simulink model "printable_simulation"  (R2024b)
settings: Solver=ode1be  StartTime=0.0  StopTime=10  FixedStep=0.001  RelTol=1e-3
model workspace (MAT data in the model file):
  AMP = 1
  FREQ = 1
  i_abc = 1
undefined symbols (not defined in the file or in its folder): Drive_wheel, Driveshaft, eff_shaft, f_OVD, i, J_S21, Jr2, K, M_curve_1, M_curve_2, M_total, mi_c, mi_s, Mode, N_clutch, n_curve_1, n_curve_2, n_max_1, n_max_2, n_surfaces, Pl, r_eq_clutch, r_geom, Shaft, sigma0, sigma1, sigma2, Spurs_Inertia, Stage1, Stage2, Stage3, vs, wheel_width
libraries: simulink x12, slpidlib x1
(part 2 of 3)

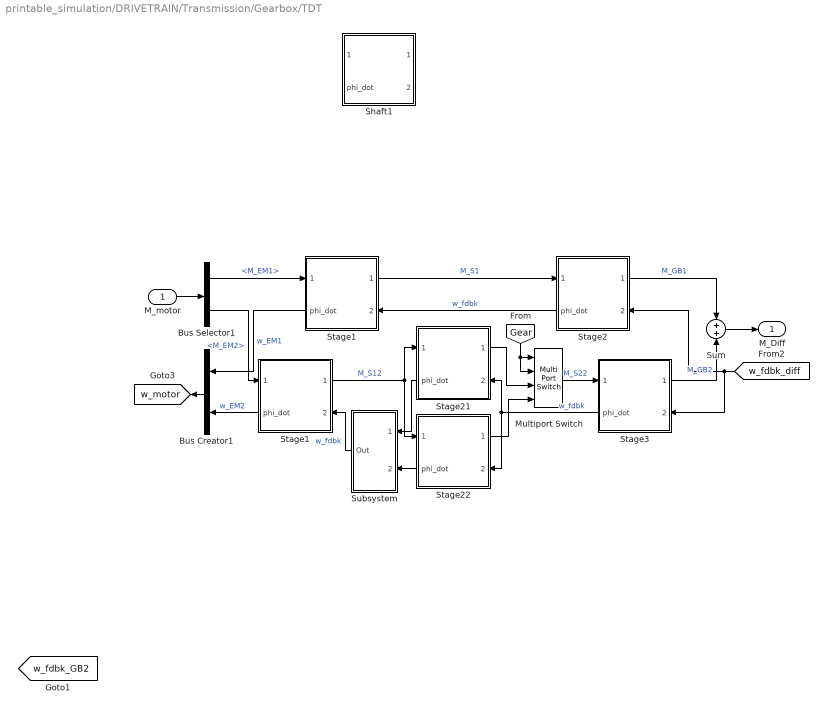
== system printable_simulation/DRIVETRAIN/Transmission/Gearbox/TDT ==
  M_motor : Inport
  Bus Creator1 : BusCreator  Inputs=2
  Bus Selector1 : BusSelector  OutputSignals=M_EM1,M_EM2
  Multiport Switch : MultiPortSwitch  DataPortOrder=Zero-based contiguous  zeroidx=on  SaturateOnIntegerOverflow=off  InputSameDT=off
  Shaft1 : Subsystem  mask{J=Shaft.J}
      mask prompts: J "Inertia_kgm^2"
      settings: PortSchema="{\"entries\":[{\"content\":{\"sides\":[{\"content\":{\"connectorIds\":[\"In1\",\"Out2\"]},\"type\":\"ConnectorPlacement.EquallySpacedRectSide\",\"uuid\":\"898fedf9-82f7-4bc2-bf05-880de36b191d\"},{\"content\":{\"connectorIds\":[\"Out1\",\"In2\"],\"side\":\"RIGHT\"},\"type\":\"ConnectorPlacement.EquallySpacedRectSide\",\"uuid\":\"50317b6c-245f-4bd1-a8cd-7a774957ae86\"},{\"content\":{\"side\":\"TOP\"},\"type\":\"ConnectorPlacement.EquallySpacedRectSide\",\"uuid\":\"ff1de2a1-7305-40d8-9e1f-fd0fa1e7d830\"}]},\"type\":\"ConnectorPlacement.EquallySpacedConnector\",\"uuid\":\"6ce82d73-f3da-4f59-9039-464a6ef3e9c5\"}],\"packageUris\":[\"http://schema.mathworks.com/mf0/Connector/R2020b\"],\"version\":\"1.0\"}"
  Stage1 : Subsystem  mask{i=Stage2.i1, J1=Stage2.Spur11.J, J2=Stage2.Spur12.J}
      mask prompts: i "Ratio"; J1 "Input_Gear_Inertia"; J2 "Output_Gear_Inertia"
      settings: PortSchema="{\"entries\":[{\"content\":{\"sides\":[{\"content\":{\"connectorIds\":[\"In1\",\"Out2\"]},\"type\":\"ConnectorPlacement.EquallySpacedRectSide\",\"uuid\":\"898fedf9-82f7-4bc2-bf05-880de36b191d\"},{\"content\":{\"connectorIds\":[\"Out1\",\"In2\"],\"side\":\"RIGHT\"},\"type\":\"ConnectorPlacement.EquallySpacedRectSide\",\"uuid\":\"50317b6c-245f-4bd1-a8cd-7a774957ae86\"},{\"content\":{\"side\":\"TOP\"},\"type\":\"ConnectorPlacement.EquallySpacedRectSide\",\"uuid\":\"ff1de2a1-7305-40d8-9e1f-fd0fa1e7d830\"}]},\"type\":\"ConnectorPlacement.EquallySpacedConnector\",\"uuid\":\"6ce82d73-f3da-4f59-9039-464a6ef3e9c5\"}],\"packageUris\":[\"http://schema.mathworks.com/mf0/Connector/R2020b\"],\"version\":\"1.0\"}"
      mask Display: image("images/spur_reduction.jpg");
  "Stage1 " : Subsystem  mask{i=Stage2.i1, J1=Stage2.Spur11.J, J2=Stage2.Spur12.J}
      mask prompts: i "Ratio"; J1 "Input_Gear_Inertia"; J2 "Output_Gear_Inertia"
      settings: PortSchema="{\"entries\":[{\"content\":{\"sides\":[{\"content\":{\"connectorIds\":[\"In1\",\"Out2\"]},\"type\":\"ConnectorPlacement.EquallySpacedRectSide\",\"uuid\":\"898fedf9-82f7-4bc2-bf05-880de36b191d\"},{\"content\":{\"connectorIds\":[\"Out1\",\"In2\"],\"side\":\"RIGHT\"},\"type\":\"ConnectorPlacement.EquallySpacedRectSide\",\"uuid\":\"50317b6c-245f-4bd1-a8cd-7a774957ae86\"},{\"content\":{\"side\":\"TOP\"},\"type\":\"ConnectorPlacement.EquallySpacedRectSide\",\"uuid\":\"ff1de2a1-7305-40d8-9e1f-fd0fa1e7d830\"}]},\"type\":\"ConnectorPlacement.EquallySpacedConnector\",\"uuid\":\"6ce82d73-f3da-4f59-9039-464a6ef3e9c5\"}],\"packageUris\":[\"http://schema.mathworks.com/mf0/Connector/R2020b\"],\"version\":\"1.0\"}"
      mask Display: image("images/spur_reduction.jpg");
  Stage2 : Subsystem  mask{i=Stage2.i1, J1=Stage2.Spur11.J, J2=Stage2.Spur12.J}
      mask prompts: i "Ratio"; J1 "Input_Gear_Inertia"; J2 "Output_Gear_Inertia"
      settings: PortSchema="{\"entries\":[{\"content\":{\"sides\":[{\"content\":{\"connectorIds\":[\"In1\",\"Out2\"]},\"type\":\"ConnectorPlacement.EquallySpacedRectSide\",\"uuid\":\"898fedf9-82f7-4bc2-bf05-880de36b191d\"},{\"content\":{\"connectorIds\":[\"Out1\",\"In2\"],\"side\":\"RIGHT\"},\"type\":\"ConnectorPlacement.EquallySpacedRectSide\",\"uuid\":\"50317b6c-245f-4bd1-a8cd-7a774957ae86\"},{\"content\":{\"side\":\"TOP\"},\"type\":\"ConnectorPlacement.EquallySpacedRectSide\",\"uuid\":\"ff1de2a1-7305-40d8-9e1f-fd0fa1e7d830\"}]},\"type\":\"ConnectorPlacement.EquallySpacedConnector\",\"uuid\":\"6ce82d73-f3da-4f59-9039-464a6ef3e9c5\"}],\"packageUris\":[\"http://schema.mathworks.com/mf0/Connector/R2020b\"],\"version\":\"1.0\"}"
      mask Display: image("images/spur_reduction.jpg");
  Stage21 : Subsystem  mask{i=Stage2.i1, J1=Stage2.Spur11.J, J2=Stage2.Spur12.J}
      mask prompts: i "Ratio"; J1 "Input_Gear_Inertia"; J2 "Output_Gear_Inertia"
      settings: PortSchema="{\"entries\":[{\"content\":{\"sides\":[{\"content\":{\"connectorIds\":[\"In1\",\"Out2\"]},\"type\":\"ConnectorPlacement.EquallySpacedRectSide\",\"uuid\":\"898fedf9-82f7-4bc2-bf05-880de36b191d\"},{\"content\":{\"connectorIds\":[\"Out1\",\"In2\"],\"side\":\"RIGHT\"},\"type\":\"ConnectorPlacement.EquallySpacedRectSide\",\"uuid\":\"50317b6c-245f-4bd1-a8cd-7a774957ae86\"},{\"content\":{\"side\":\"TOP\"},\"type\":\"ConnectorPlacement.EquallySpacedRectSide\",\"uuid\":\"ff1de2a1-7305-40d8-9e1f-fd0fa1e7d830\"}]},\"type\":\"ConnectorPlacement.EquallySpacedConnector\",\"uuid\":\"6ce82d73-f3da-4f59-9039-464a6ef3e9c5\"}],\"packageUris\":[\"http://schema.mathworks.com/mf0/Connector/R2020b\"],\"version\":\"1.0\"}"
      mask Display: image("images/spur_reduction.jpg");
  Stage22 : Subsystem  mask{i=Stage2.i1, J1=Stage2.Spur11.J, J2=Stage2.Spur12.J}
      mask prompts: i "Ratio"; J1 "Input_Gear_Inertia"; J2 "Output_Gear_Inertia"
      settings: PortSchema="{\"entries\":[{\"content\":{\"sides\":[{\"content\":{\"connectorIds\":[\"In1\",\"Out2\"]},\"type\":\"ConnectorPlacement.EquallySpacedRectSide\",\"uuid\":\"898fedf9-82f7-4bc2-bf05-880de36b191d\"},{\"content\":{\"connectorIds\":[\"Out1\",\"In2\"],\"side\":\"RIGHT\"},\"type\":\"ConnectorPlacement.EquallySpacedRectSide\",\"uuid\":\"50317b6c-245f-4bd1-a8cd-7a774957ae86\"},{\"content\":{\"side\":\"TOP\"},\"type\":\"ConnectorPlacement.EquallySpacedRectSide\",\"uuid\":\"ff1de2a1-7305-40d8-9e1f-fd0fa1e7d830\"}]},\"type\":\"ConnectorPlacement.EquallySpacedConnector\",\"uuid\":\"6ce82d73-f3da-4f59-9039-464a6ef3e9c5\"}],\"packageUris\":[\"http://schema.mathworks.com/mf0/Connector/R2020b\"],\"version\":\"1.0\"}"
      mask Display: image("images/spur_reduction.jpg");
  Stage3 : Subsystem  mask{i=Stage2.i1, J1=Stage2.Spur11.J, J2=Stage2.Spur12.J}
      mask prompts: i "Ratio"; J1 "Input_Gear_Inertia"; J2 "Output_Gear_Inertia"
      settings: PortSchema="{\"entries\":[{\"content\":{\"sides\":[{\"content\":{\"connectorIds\":[\"In1\",\"Out2\"]},\"type\":\"ConnectorPlacement.EquallySpacedRectSide\",\"uuid\":\"898fedf9-82f7-4bc2-bf05-880de36b191d\"},{\"content\":{\"connectorIds\":[\"Out1\",\"In2\"],\"side\":\"RIGHT\"},\"type\":\"ConnectorPlacement.EquallySpacedRectSide\",\"uuid\":\"50317b6c-245f-4bd1-a8cd-7a774957ae86\"},{\"content\":{\"side\":\"TOP\"},\"type\":\"ConnectorPlacement.EquallySpacedRectSide\",\"uuid\":\"ff1de2a1-7305-40d8-9e1f-fd0fa1e7d830\"}]},\"type\":\"ConnectorPlacement.EquallySpacedConnector\",\"uuid\":\"6ce82d73-f3da-4f59-9039-464a6ef3e9c5\"}],\"packageUris\":[\"http://schema.mathworks.com/mf0/Connector/R2020b\"],\"version\":\"1.0\"}"
      mask Display: image("images/spur_reduction.jpg");
  Subsystem : Subsystem
      settings: PortSchema="{\"entries\":[{\"content\":{\"sides\":[{\"content\":{\"connectorIds\":[\"Out1\"]},\"type\":\"ConnectorPlacement.EquallySpacedRectSide\",\"uuid\":\"fb6fb521-24b4-42a9-962b-0690c95a6555\"},{\"content\":{\"connectorIds\":[\"In1\",\"In2\"],\"side\":\"RIGHT\"},\"type\":\"ConnectorPlacement.EquallySpacedRectSide\",\"uuid\":\"05ff3728-9142-4ede-8c02-c3816594f1d6\"},{\"content\":{\"side\":\"TOP\"},\"type\":\"ConnectorPlacement.EquallySpacedRectSide\",\"uuid\":\"6bf5bb06-bb76-41b4-800b-6d1bd3df4c7c\"}]},\"type\":\"ConnectorPlacement.EquallySpacedConnector\",\"uuid\":\"4f0648fe-100b-4dfa-b2f8-0696c3f6a986\"}],\"packageUris\":[\"http://schema.mathworks.com/mf0/Connector/R2020b\"],\"version\":\"1.0\"}"
      mask Display: image("images/switch.png");
  Sum : Sum  Inputs=+|+
  M_Diff : Outport
  tag scope: w_fdbk_GB2=global, w_motor=global
  wires:
  "Stage1 "/1(Torque_out) -> Stage21/1(Torque_in), Stage22/1(Torque_in)  "M_S12"
  M_motor/1 -> Bus Selector1/1
  Stage3/1(Torque_out) -> Sum/2  "M_GB2"
  Bus Selector1/1 -> Stage1/1(Torque_in)  "<M_EM1>"
  Stage2/1(Torque_out) -> Sum/1  "M_GB1"
  Stage1/2(phi_dot) -> Bus Creator1/1  "w_EM1"
  Bus Selector1/2 -> "Stage1 "/1(Torque_in)  "<M_EM2>"
  Sum/1 -> M_Diff/1
  Stage1/1(Torque_out) -> Stage2/1(Torque_in)  "M_S1"
  Stage3/2(phi_dot) -> Stage22/2(Speed_fdbk), Stage21/2(Speed_fdbk)  "w_fdbk"
  Multiport Switch/1 -> Stage3/1(Torque_in)  "M_S22"
  Stage22/2(phi_dot) -> Subsystem/2(Spur22)
  [w_fdbk_diff] -> Stage2/2(Speed_fdbk), Stage3/2(Speed_fdbk)
  Stage22/1(Torque_out) -> Multiport Switch/4
  [Gear] -> Multiport Switch/1, Multiport Switch/2
  Stage21/2(phi_dot) -> Subsystem/1(Spur 21)
  "Stage1 "/2(phi_dot) -> Bus Creator1/2  "w_EM2"
  Bus Creator1/1 -> [w_motor]
  Stage21/1(Torque_out) -> Multiport Switch/3
  Stage2/2(phi_dot) -> Stage1/2(Speed_fdbk)  "w_fdbk"
  Subsystem/1(Out) -> "Stage1 "/2(Speed_fdbk)  "w_fdbk"

== system printable_simulation/DRIVETRAIN/Transmission/Gearbox/e-CVT ==
  M_motor : Inport
  M_Diff : Outport
  wires:
  M_motor/1 -> M_Diff/1

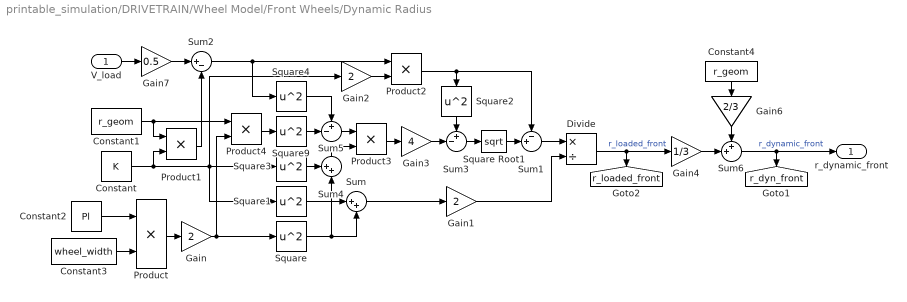
== system printable_simulation/DRIVETRAIN/Wheel Model/Front Wheels/Dynamic Radius ==
  V_load : Inport
  Constant : Constant  Value=K
  Constant1 : Constant  Value=r_geom
  Constant2 : Constant  Value=Pl
  Constant3 : Constant  Value=wheel_width
  Constant4 : Constant  Value=r_geom
  Divide : Product  Inputs=*/
  Gain : Gain  Gain=2
  Gain1 : Gain  Gain=2
  Gain2 : Gain  Gain=2
  Gain3 : Gain  Gain=4
  Gain4 : Gain  Gain=1/3
  Gain6 : Gain  Gain=2/3
  Gain7 : Gain  Gain=0.5
  Product{,1..4} (5 alike) : Product
  Square{,1..4,9} (6 alike) : Math  Operator=square
  Square Root1 : Sqrt
  Sum : Sum  Inputs=|++
  Sum1 : Sum  Inputs=-+|
  Sum2 : Sum  Inputs=|+-
  Sum3 : Sum  Inputs=+-|
  Sum4 : Sum  Inputs=++|
  Sum5 : Sum  Inputs=+-|
  Sum6 : Sum  Inputs=++|
  r_dynamic_front : Outport
  tag scope: r_dyn_front=global, r_loaded_front=global
  wires:
  Square1/1 -> Sum/1
  Divide/1 -> Gain4/1, [r_loaded_front]  "r_loaded_front"
  Square3/1 -> Sum4/1
  Sum/1 -> Gain1/1
  Sum1/1 -> Divide/1
  Constant/1 -> Product1/2, Square3/1, Gain2/1, Square1/1
  Constant3/1 -> Product/2
  Product1/1 -> Sum2/2
  Square Root1/1 -> Sum1/2
  Gain3/1 -> Sum3/2
  Gain/1 -> Product4/2, Square/1
  Constant2/1 -> Product/1
  Sum5/1 -> Product3/1
  Product3/1 -> Gain3/1
  Gain1/1 -> Divide/2
  Constant1/1 -> Product4/1, Product1/1
  Square9/1 -> Sum5/2
  Square/1 -> Sum4/2, Sum/2
  Sum4/1 -> Product3/2
  Sum3/1 -> Square Root1/1
  Square4/1 -> Sum5/1
  Sum2/1 -> Square4/1, Product2/1
  Product4/1 -> Square9/1
  Product/1 -> Gain/1
  Square2/1 -> Sum3/1
  Gain4/1 -> Sum6/2
  Gain6/1 -> Sum6/1
  Gain7/1 -> Sum2/1
  Constant4/1 -> Gain6/1
  Gain2/1 -> Product2/2
  Sum6/1 -> r_dynamic_front/1, [r_dyn_front]  "r_dynamic_front"
  Product2/1 -> Square2/1, Sum1/1
  V_load/1 -> Gain7/1

== system printable_simulation/DRIVETRAIN/Wheel Model/Front Wheels/Wheel Torque ==
  M_tra : Inport
  M_break : Inport  Port=2
  Bus Selector1 : BusSelector  OutputSignals=M_axleL,M_axleR
  Constant5 : Constant  Value=Drive_wheel
  Gain9 : Gain  Gain=0.5
  Multiport Switch : MultiPortSwitch  DataPortOrder=Zero-based contiguous  zeroidx=on  SaturateOnIntegerOverflow=off  InputSameDT=off
  Sum3 : Sum  Inputs=++|
  Sum4 : Sum  Inputs=++|
  Sum8 : Sum  Inputs=+|+
  M_front_wheels : Outport
  tag scope: M_front_wheels=global
  wires:
  Multiport Switch/1 -> M_front_wheels/1, [M_front_wheels]  "M_front_wheels"
  Bus Selector1/1 -> Sum8/1  "<M_axleL>"
  Constant5/1 -> Multiport Switch/1
  Gain9/1 -> Sum3/2
  M_break/1 -> Sum4/1, Sum3/1, Multiport Switch/2
  Bus Selector1/2 -> Sum8/2  "<M_axleR>"
  M_tra/1 -> Bus Selector1/1
  Sum8/1 -> Sum4/2, Gain9/1
  Sum3/1 -> Multiport Switch/4
  Sum4/1 -> Multiport Switch/3

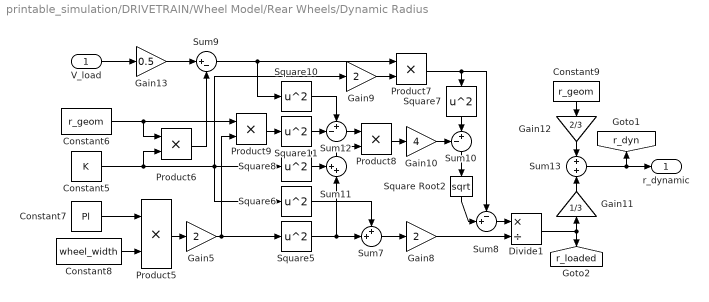
== system printable_simulation/DRIVETRAIN/Wheel Model/Rear Wheels/Dynamic Radius ==
  V_load : Inport
  Constant5 : Constant  Value=K
  Constant6 : Constant  Value=r_geom
  Constant7 : Constant  Value=Pl
  Constant8 : Constant  Value=wheel_width
  Constant9 : Constant  Value=r_geom
  Divide1 : Product  Inputs=*/
  Gain10 : Gain  Gain=4
  Gain11 : Gain  Gain=1/3
  Gain12 : Gain  Gain=2/3
  Gain13 : Gain  Gain=0.5
  Gain5 : Gain  Gain=2
  Gain8 : Gain  Gain=2
  Gain9 : Gain  Gain=2
  Product{5..9} (5 alike) : Product
  Square Root2 : Sqrt
  Square{5..8,10..11} (6 alike) : Math  Operator=square
  Sum10 : Sum  Inputs=-+|
  Sum11 : Sum  Inputs=++|
  Sum12 : Sum  Inputs=+-|
  Sum13 : Sum  Inputs=+|+
  Sum7 : Sum  Inputs=++|
  Sum8 : Sum  Inputs=-+|
  Sum9 : Sum  Inputs=|+-
  r_dynamic : Outport
  tag scope: r_dyn=global, r_loaded=global
  wires:
  Gain11/1 -> Sum13/2
  Square Root2/1 -> Sum8/2
  Gain9/1 -> Product7/2
  Gain10/1 -> Sum10/1
  Constant8/1 -> Product5/2
  Gain5/1 -> Square5/1, Product9/2
  Gain13/1 -> Sum9/1
  Sum12/1 -> Product8/1
  Product5/1 -> Gain5/1
  Product7/1 -> Sum8/1, Square7/1
  Constant6/1 -> Product9/1, Product6/1
  V_load/1 -> Gain13/1
  Gain8/1 -> Divide1/2
  Square11/1 -> Sum12/2
  Sum10/1 -> Square Root2/1
  Sum9/1 -> Product7/1, Square10/1
  Gain12/1 -> Sum13/1
  Square6/1 -> Sum7/1
  Divide1/1 -> Gain11/1, [r_loaded]
  Sum13/1 -> r_dynamic/1, [r_dyn]
  Product8/1 -> Gain10/1
  Constant9/1 -> Gain12/1
  Sum7/1 -> Gain8/1
  Product6/1 -> Sum9/2
  Square5/1 -> Sum11/2, Sum7/2
  Sum11/1 -> Product8/2
  Square8/1 -> Sum11/1
  Sum8/1 -> Divide1/1
  Constant5/1 -> Square6/1, Gain9/1, Square8/1, Product6/2
  Product9/1 -> Square11/1
  Constant7/1 -> Product5/1
  Square10/1 -> Sum12/1
  Square7/1 -> Sum10/2

== system printable_simulation/DRIVETRAIN/Wheel Model/Rear Wheels/Wheel Torque ==
  M_tra : Inport
  M_break : Inport  Port=2
  Bus Selector1 : BusSelector  OutputSignals=M_axleL,M_axleR
  Constant5 : Constant  Value=Drive_wheel
  Gain : Gain  Gain=0.5
  Multiport Switch : MultiPortSwitch  DataPortOrder=Zero-based contiguous  zeroidx=on  SaturateOnIntegerOverflow=off  InputSameDT=off
  Sum : Sum  Inputs=|++
  Sum1 : Sum  Inputs=++|
  Sum8 : Sum  Inputs=+|+
  M_rear_wheels : Outport
  tag scope: M_rear_wheels=global
  wires:
  Multiport Switch/1 -> [M_rear_wheels], M_rear_wheels/1  "M_rear_wheels"
  Sum8/1 -> Gain/1, Sum/1
  Sum/1 -> Multiport Switch/2
  M_break/1 -> Sum/2, Sum1/1, Multiport Switch/3
  Bus Selector1/1 -> Sum8/1  "<M_axleL>"
  Bus Selector1/2 -> Sum8/2  "<M_axleR>"
  Constant5/1 -> Multiport Switch/1
  M_tra/1 -> Bus Selector1/1
  Gain/1 -> Sum1/2
  Sum1/1 -> Multiport Switch/4

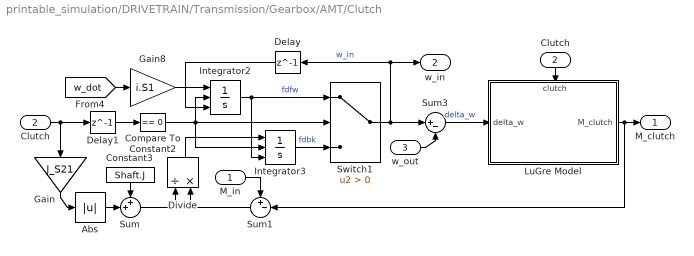
== system printable_simulation/DRIVETRAIN/Transmission/Gearbox/AMT/Clutch ==
  M_in : Inport
  "Clutch " : Inport  Port=2
  w_out : Inport  Port=3
  " Clutch  " : InportShadow  Port=2
  Abs : Abs  SaturateOnIntegerOverflow=off
  Compare To Constant2 : simulink/Logic and Bit Operations/Compare To Constant  relop===  const=0  OutDataTypeStr=boolean
  Constant3 : Constant  Value=Shaft.J
  Delay : Delay  DelayLength=1  InputProcessing=Columns as channels (frame based)
  Delay1 : Delay  DelayLength=1  InputProcessing=Columns as channels (frame based)
  Divide : Product  Inputs=/*
  Gain : Gain  Gain=J_S21
  Gain8 : Gain  Gain=i.S1
  Integrator2 : Integrator  ExternalReset=either  InitialConditionSource=external
  Integrator3 : Integrator  ExternalReset=either  InitialConditionSource=external
  LuGre Model : Subsystem
      settings: PortSchema="{\"entries\":[{\"content\":{\"sides\":[{\"content\":{\"connectorIds\":[\"In1\"]},\"type\":\"ConnectorPlacement.EquallySpacedRectSide\",\"uuid\":\"a26f5a32-9f9c-4306-b7a8-6355090a4a86\"},{\"content\":{\"connectorIds\":[\"Out1\"],\"side\":\"RIGHT\"},\"type\":\"ConnectorPlacement.EquallySpacedRectSide\",\"uuid\":\"4fa489e2-cd1d-4a36-b0cb-261100046200\"},{\"content\":{\"connectorIds\":[\"In2\"],\"side\":\"TOP\"},\"type\":\"ConnectorPlacement.EquallySpacedRectSide\",\"uuid\":\"0e05a540-d6e3-4351-9a32-83f6c32571ff\"}]},\"type\":\"ConnectorPlacement.EquallySpacedConnector\",\"uuid\":\"492e0439-728a-4999-b29b-e2639b0e762e\"}],\"packageUris\":[\"http://schema.mathworks.com/mf0/Connector/R2020b\"],\"version\":\"1.0\"}"
      mask Display: image('images/Elastic_bristles.png');
  Sum : Sum  Inputs=++|
  Sum1 : Sum  Inputs=+-|
  Sum3 : Sum  Inputs=|+-
  Switch1 : Switch  Criteria=u2 > Threshold  SaturateOnIntegerOverflow=off  InputSameDT=off
  M_clutch : Outport
  w_in : Outport  Port=2
  wires:
  Switch1/1 -> Delay/1, w_in/1, Sum3/1  "w_in"
  Sum3/1 -> LuGre Model/1(delta_w)  "delta_w"
  Sum/1 -> Divide/1
  M_in/1 -> Sum1/1
  Constant3/1 -> Sum/1
  w_out/1 -> Sum3/2
  Gain/1 -> Abs/1
  LuGre Model/1(M_clutch) -> M_clutch/1, Sum1/2
  Sum1/1 -> Divide/2
  Divide/1 -> Integrator3/1
  Gain8/1 -> Integrator2/1
  Integrator2/1 -> Switch1/1, Integrator3/3  "fdfw"
  [w_dot] -> Gain8/1
  Compare To Constant2/1 -> Integrator3/2, Integrator2/2, Switch1/2
  Delay/1 -> Integrator2/3
  Integrator3/1 -> Switch1/3  "fdbk"
  "Clutch "/1 -> Delay1/1, Gain/1
  Delay1/1 -> Compare To Constant2/1
  " Clutch  "/1 -> LuGre Model/2(" clutch")
  Abs/1 -> Sum/2

== system printable_simulation/DRIVETRAIN/Transmission/Gearbox/AMT/Stage1 ==
  Torque_in : Inport
  Speed_fdbk : Inport  Port=2
  Derivative : Derivative
  Derivative1 : Derivative
  Gain : Gain  Gain=i
  Gain2 : Gain  Gain=J2
  Gain3 : Gain  Gain=J1
  Gain4 : Gain  Gain=i
  Sum1 : Sum  Inputs=|+-
  Sum2 : Sum  Inputs=|+-
  Torque_out : Outport
  phi_dot : Outport  Port=2
  wires:
  Derivative/1 -> Gain2/1
  Derivative1/1 -> Gain3/1
  Sum1/1 -> Gain/1
  Gain2/1 -> Sum2/2
  Speed_fdbk/1 -> Derivative/1, Gain4/1
  Gain4/1 -> phi_dot/1, Derivative1/1
  Torque_in/1 -> Sum1/1
  Gain3/1 -> Sum1/2
  Sum2/1 -> Torque_out/1
  Gain/1 -> Sum2/1

== system printable_simulation/DRIVETRAIN/Transmission/Gearbox/AMT/Stage21 ==
  Torque_in : Inport
  Speed_fdbk : Inport  Port=2
  Derivative : Derivative
  Derivative1 : Derivative
  Gain : Gain  Gain=i
  Gain2 : Gain  Gain=J2
  Gain3 : Gain  Gain=J1
  Gain4 : Gain  Gain=i
  Sum1 : Sum  Inputs=|+-
  Sum2 : Sum  Inputs=|+-
  Torque_out : Outport
  phi_dot : Outport  Port=2
  wires:
  Gain/1 -> Sum2/1
  Sum2/1 -> Torque_out/1
  Gain3/1 -> Sum1/2
  Torque_in/1 -> Sum1/1
  Gain4/1 -> Derivative1/1, phi_dot/1
  Speed_fdbk/1 -> Gain4/1, Derivative/1
  Gain2/1 -> Sum2/2
  Sum1/1 -> Gain/1
  Derivative1/1 -> Gain3/1
  Derivative/1 -> Gain2/1

== system printable_simulation/DRIVETRAIN/Transmission/Gearbox/AMT/Stage22 ==
  Torque_in : Inport
  Speed_fdbk : Inport  Port=2
  Derivative : Derivative
  Derivative1 : Derivative
  Gain : Gain  Gain=i
  Gain2 : Gain  Gain=J2
  Gain3 : Gain  Gain=J1
  Gain4 : Gain  Gain=i
  Sum1 : Sum  Inputs=|+-
  Sum2 : Sum  Inputs=|+-
  Torque_out : Outport
  phi_dot : Outport  Port=2
  wires:
  Derivative/1 -> Gain2/1
  Derivative1/1 -> Gain3/1
  Sum1/1 -> Gain/1
  Gain2/1 -> Sum2/2
  Speed_fdbk/1 -> Derivative/1, Gain4/1
  Gain4/1 -> phi_dot/1, Derivative1/1
  Torque_in/1 -> Sum1/1
  Gain3/1 -> Sum1/2
  Sum2/1 -> Torque_out/1
  Gain/1 -> Sum2/1

== system printable_simulation/DRIVETRAIN/Transmission/Gearbox/AMT/Stage3 ==
  Torque_in : Inport
  Speed_fdbk : Inport  Port=2
  Derivative : Derivative
  Derivative1 : Derivative
  Gain : Gain  Gain=i
  Gain2 : Gain  Gain=J2
  Gain3 : Gain  Gain=J1
  Gain4 : Gain  Gain=i
  Sum1 : Sum  Inputs=|+-
  Sum2 : Sum  Inputs=|+-
  Torque_out : Outport
  phi_dot : Outport  Port=2
  wires:
  Derivative/1 -> Gain2/1
  Derivative1/1 -> Gain3/1
  Sum1/1 -> Gain/1
  Gain2/1 -> Sum2/2
  Speed_fdbk/1 -> Derivative/1, Gain4/1
  Gain4/1 -> phi_dot/1, Derivative1/1
  Torque_in/1 -> Sum1/1
  Gain3/1 -> Sum1/2
  Sum2/1 -> Torque_out/1
  Gain/1 -> Sum2/1

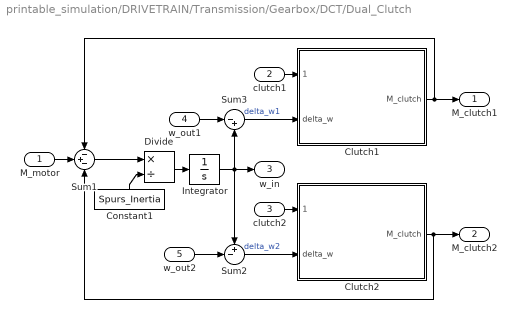
== system printable_simulation/DRIVETRAIN/Transmission/Gearbox/DCT/Dual_Clutch ==
  M_motor : Inport
  clutch1 : Inport  Port=2
  clutch2 : Inport  Port=3
  w_out1 : Inport  Port=4
  w_out2 : Inport  Port=5
  Clutch1 : Subsystem
      mask Display: image('images/Elastic_bristles.png')
  Clutch2 : Subsystem
      mask Display: image('images/Elastic_bristles.png')
  Constant1 : Constant  Value=Spurs_Inertia
  Divide : Product  Inputs=*/
  Integrator : Integrator
  Sum1 : Sum  Inputs=-+-
  Sum2 : Sum  Inputs=+-|
  Sum3 : Sum  Inputs=|-+
  M_clutch1 : Outport
  M_clutch2 : Outport  Port=2
  w_in : Outport  Port=3
  wires:
  Sum3/1 -> Clutch1/2(delta_w)  "delta_w1"
  M_motor/1 -> Sum1/2
  w_out1/1 -> Sum3/1
  Clutch1/1(M_clutch) -> Sum1/1, M_clutch1/1
  Sum1/1 -> Divide/1
  clutch1/1 -> Clutch1/1(" ")
  Integrator/1 -> w_in/1, Sum2/1, Sum3/2
  Clutch2/1(M_clutch) -> M_clutch2/1, Sum1/3
  clutch2/1 -> Clutch2/1(" ")
  w_out2/1 -> Sum2/2
  Sum2/1 -> Clutch2/2(delta_w)  "delta_w2"
  Divide/1 -> Integrator/1
  Constant1/1 -> Divide/2

== system printable_simulation/DRIVETRAIN/Transmission/Gearbox/DCT/Stage_2.1 ==
  note: 1) Add Subsystem or Model blocks as valid variant choices.
      | 2) You cannot connect blocks at this level. At simulation, connectivity is automatically
      | determined, based on the active variant and port name matching.
  Torque_in : Inport
  Speed_fdbk : Inport  Port=2
  Nothing : Subsystem  VariantControl=Stage2.Type == 0
  Spur : Subsystem  VariantControl=Stage2.Type == 1
  Torque_out : Outport
  Speed_out : Outport  Port=2

== system printable_simulation/DRIVETRAIN/Transmission/Gearbox/DCT/Stage_2.2 ==
  note: 1) Add Subsystem or Model blocks as valid variant choices.
      | 2) You cannot connect blocks at this level. At simulation, connectivity is automatically
      | determined, based on the active variant and port name matching.
  Torque_in : Inport
  Speed_fdbk : Inport  Port=2
  Nothing : Subsystem  VariantControl=Stage2.Type == 0
  Spur : Subsystem  VariantControl=Stage2.Type == 1
  Torque_out : Outport
  Speed_out : Outport  Port=2

== system printable_simulation/DRIVETRAIN/Transmission/Gearbox/DCT/Stage_3 ==
  note: 1) Add Subsystem or Model blocks as valid variant choices.
      | 2) You cannot connect blocks at this level. At simulation, connectivity is automatically
      | determined, based on the active variant and port name matching.
  Torque_in : Inport
  Speed_fdbk : Inport  Port=2
  Nothing : Subsystem  VariantControl=Stage3.Type == 0
  Spur : Subsystem  VariantControl=Stage3.Type == 1
  Torque_out : Outport
  Speed_out : Outport  Port=2

== system printable_simulation/DRIVETRAIN/Transmission/Gearbox/TDT/Shaft1 ==
  Torque_in : Inport
  Speed_fdbk : Inport  Port=2
  Derivative : Derivative
  Gain3 : Gain  Gain=J
  Sum1 : Sum  Inputs=|+-
  Torque_out : Outport
  phi_dot : Outport  Port=2
  wires:
  Torque_in/1 -> Sum1/1
  Gain3/1 -> Sum1/2
  Derivative/1 -> Gain3/1
  Sum1/1 -> Torque_out/1
  Speed_fdbk/1 -> Derivative/1, phi_dot/1

== system printable_simulation/DRIVETRAIN/Transmission/Gearbox/TDT/Stage1 ==
  Torque_in : Inport
  Speed_fdbk : Inport  Port=2
  Derivative : Derivative
  Derivative1 : Derivative
  Gain : Gain  Gain=i
  Gain2 : Gain  Gain=J2
  Gain3 : Gain  Gain=J1
  Gain4 : Gain  Gain=i
  Sum1 : Sum  Inputs=|+-
  Sum2 : Sum  Inputs=|+-
  Torque_out : Outport
  phi_dot : Outport  Port=2
  wires:
  Gain/1 -> Sum2/1
  Sum2/1 -> Torque_out/1
  Gain3/1 -> Sum1/2
  Torque_in/1 -> Sum1/1
  Gain4/1 -> Derivative1/1, phi_dot/1
  Speed_fdbk/1 -> Gain4/1, Derivative/1
  Gain2/1 -> Sum2/2
  Sum1/1 -> Gain/1
  Derivative1/1 -> Gain3/1
  Derivative/1 -> Gain2/1

== system printable_simulation/DRIVETRAIN/Transmission/Gearbox/TDT/Stage1  ==
  Torque_in : Inport
  Speed_fdbk : Inport  Port=2
  Derivative : Derivative
  Derivative1 : Derivative
  Gain : Gain  Gain=i
  Gain2 : Gain  Gain=J2
  Gain3 : Gain  Gain=J1
  Gain4 : Gain  Gain=i
  Sum1 : Sum  Inputs=|+-
  Sum2 : Sum  Inputs=|+-
  Torque_out : Outport
  phi_dot : Outport  Port=2
  wires:
  Derivative/1 -> Gain2/1
  Derivative1/1 -> Gain3/1
  Sum1/1 -> Gain/1
  Gain2/1 -> Sum2/2
  Speed_fdbk/1 -> Derivative/1, Gain4/1
  Gain4/1 -> phi_dot/1, Derivative1/1
  Torque_in/1 -> Sum1/1
  Gain3/1 -> Sum1/2
  Sum2/1 -> Torque_out/1
  Gain/1 -> Sum2/1

== system printable_simulation/DRIVETRAIN/Transmission/Gearbox/TDT/Stage2 ==
  Torque_in : Inport
  Speed_fdbk : Inport  Port=2
  Derivative : Derivative
  Derivative1 : Derivative
  Gain : Gain  Gain=i
  Gain2 : Gain  Gain=J2
  Gain3 : Gain  Gain=J1
  Gain4 : Gain  Gain=i
  Sum1 : Sum  Inputs=|+-
  Sum2 : Sum  Inputs=|+-
  Torque_out : Outport
  phi_dot : Outport  Port=2
  wires:
  Derivative/1 -> Gain2/1
  Derivative1/1 -> Gain3/1
  Sum1/1 -> Gain/1
  Gain2/1 -> Sum2/2
  Speed_fdbk/1 -> Derivative/1, Gain4/1
  Gain4/1 -> phi_dot/1, Derivative1/1
  Torque_in/1 -> Sum1/1
  Gain3/1 -> Sum1/2
  Sum2/1 -> Torque_out/1
  Gain/1 -> Sum2/1

== system printable_simulation/DRIVETRAIN/Transmission/Gearbox/TDT/Stage21 ==
  Torque_in : Inport
  Speed_fdbk : Inport  Port=2
  Derivative : Derivative
  Derivative1 : Derivative
  Gain : Gain  Gain=i
  Gain2 : Gain  Gain=J2
  Gain3 : Gain  Gain=J1
  Gain4 : Gain  Gain=i
  Sum1 : Sum  Inputs=|+-
  Sum2 : Sum  Inputs=|+-
  Torque_out : Outport
  phi_dot : Outport  Port=2
  wires:
  Derivative/1 -> Gain2/1
  Derivative1/1 -> Gain3/1
  Sum1/1 -> Gain/1
  Gain2/1 -> Sum2/2
  Speed_fdbk/1 -> Derivative/1, Gain4/1
  Gain4/1 -> phi_dot/1, Derivative1/1
  Torque_in/1 -> Sum1/1
  Gain3/1 -> Sum1/2
  Sum2/1 -> Torque_out/1
  Gain/1 -> Sum2/1

== system printable_simulation/DRIVETRAIN/Transmission/Gearbox/TDT/Stage22 ==
  Torque_in : Inport
  Speed_fdbk : Inport  Port=2
  Derivative : Derivative
  Derivative1 : Derivative
  Gain : Gain  Gain=i
  Gain2 : Gain  Gain=J2
  Gain3 : Gain  Gain=J1
  Gain4 : Gain  Gain=i
  Sum1 : Sum  Inputs=|+-
  Sum2 : Sum  Inputs=|+-
  Torque_out : Outport
  phi_dot : Outport  Port=2
  wires:
  Derivative/1 -> Gain2/1
  Derivative1/1 -> Gain3/1
  Sum1/1 -> Gain/1
  Gain2/1 -> Sum2/2
  Speed_fdbk/1 -> Derivative/1, Gain4/1
  Gain4/1 -> phi_dot/1, Derivative1/1
  Torque_in/1 -> Sum1/1
  Gain3/1 -> Sum1/2
  Sum2/1 -> Torque_out/1
  Gain/1 -> Sum2/1

== system printable_simulation/DRIVETRAIN/Transmission/Gearbox/TDT/Stage3 ==
  Torque_in : Inport
  Speed_fdbk : Inport  Port=2
  Derivative : Derivative
  Derivative1 : Derivative
  Gain : Gain  Gain=i
  Gain2 : Gain  Gain=J2
  Gain3 : Gain  Gain=J1
  Gain4 : Gain  Gain=i
  Sum1 : Sum  Inputs=|+-
  Sum2 : Sum  Inputs=|+-
  Torque_out : Outport
  phi_dot : Outport  Port=2
  wires:
  Gain/1 -> Sum2/1
  Sum2/1 -> Torque_out/1
  Gain3/1 -> Sum1/2
  Torque_in/1 -> Sum1/1
  Gain4/1 -> Derivative1/1, phi_dot/1
  Speed_fdbk/1 -> Gain4/1, Derivative/1
  Gain2/1 -> Sum2/2
  Sum1/1 -> Gain/1
  Derivative1/1 -> Gain3/1
  Derivative/1 -> Gain2/1

== system printable_simulation/DRIVETRAIN/Transmission/Gearbox/TDT/Subsystem ==
  Spur 21 : Inport
  Spur22 : Inport  Port=2
  Multiport Switch : MultiPortSwitch  DataPortOrder=Zero-based contiguous  Inputs=8  zeroidx=on  SaturateOnIntegerOverflow=off  InputSameDT=off
  Multiport Switch1 : MultiPortSwitch  DataPortOrder=Zero-based contiguous  zeroidx=on  SaturateOnIntegerOverflow=off  InputSameDT=off
  Switch : Switch  Criteria=u2 > Threshold  Threshold=1  SaturateOnIntegerOverflow=off  InputSameDT=off
  Switch1 : Switch  Criteria=u2 > Threshold  Threshold=1  SaturateOnIntegerOverflow=off  InputSameDT=off
  Out : Outport
  wires:
  Multiport Switch/1 -> Out/1
  [Gear] -> Multiport Switch1/1
  Spur 21/1 -> Multiport Switch1/3, Switch1/1, Switch/3
  Spur22/1 -> Switch/1, Switch1/3, Multiport Switch1/4
  Multiport Switch1/1 -> Multiport Switch/9, Multiport Switch/8, Multiport Switch/7, Multiport Switch/4, Multiport Switch/3, Multiport Switch/2
  [shifting_stage] -> Multiport Switch/1
  [GearSet] -> Switch/2, Switch1/2
  Switch/1 -> Multiport Switch1/2, Multiport Switch/6
  Switch1/1 -> Multiport Switch/5

== system printable_simulation/DRIVETRAIN/Transmission/Gearbox/AMT/Clutch/LuGre Model ==
  delta_w : Inport
  " clutch" : Inport  Port=2
  Gain10 : Gain  Gain=r_eq_clutch
  Gain3 : Gain  Gain=r_eq_clutch
  Subsystem : Subsystem
      settings: PortSchema="{\"entries\":[{\"content\":{\"sides\":[{\"content\":{\"connectorIds\":[\"In1\"]},\"type\":\"ConnectorPlacement.EquallySpacedRectSide\",\"uuid\":\"0ae2ed28-5be6-4ce0-b87c-2c13a72d1ad0\"},{\"content\":{\"connectorIds\":[\"In2\",\"Out1\"],\"side\":\"RIGHT\"},\"type\":\"ConnectorPlacement.EquallySpacedRectSide\",\"uuid\":\"8d48d664-ebaf-4c3e-be9e-f793543e8061\"},{\"content\":{\"side\":\"TOP\"},\"type\":\"ConnectorPlacement.EquallySpacedRectSide\",\"uuid\":\"2d66836a-de46-4974-a48b-ee2778be1c08\"},{\"content\":{\"side\":\"BOTTOM\"},\"type\":\"ConnectorPlacement.EquallySpacedRectSide\",\"uuid\":\"e232d9f4-6257-4976-8384-26c462ae0041\"}]},\"type\":\"ConnectorPlacement.EquallySpacedConnector\",\"uuid\":\"ae24f926-3a59-4a74-9cf0-af55dcfbad19\"}],\"packageUris\":[\"http://schema.mathworks.com/mf0/Connector/R2020b\"],\"version\":\"1.0\"}"
      mask Display: image('images/Stribeck.png');
  Subsystem1 : Subsystem
      settings: PortSchema="{\"entries\":[{\"content\":{\"sides\":[{\"content\":{\"connectorIds\":[\"In1\",\"In2\"]},\"type\":\"ConnectorPlacement.EquallySpacedRectSide\",\"uuid\":\"9e2cbd08-5b8a-4c75-ae53-c0d295cfe494\"},{\"content\":{\"connectorIds\":[\"Out1\",\"Out2\"],\"side\":\"RIGHT\"},\"type\":\"ConnectorPlacement.EquallySpacedRectSide\",\"uuid\":\"77a3a6f0-22a7-43a6-8d61-33ee07a6a335\"},{\"content\":{\"side\":\"TOP\"},\"type\":\"ConnectorPlacement.EquallySpacedRectSide\",\"uuid\":\"42262743-4dc6-4297-a012-95f629a18d23\"},{\"content\":{\"connectorIds\":[\"In3\"],\"side\":\"BOTTOM\"},\"type\":\"ConnectorPlacement.EquallySpacedRectSide\",\"uuid\":\"a89123f6-acee-411d-93c1-3b5d847486f5\"}]},\"type\":\"ConnectorPlacement.EquallySpacedConnector\",\"uuid\":\"ae5ede95-cba8-4d2e-b0da-ab555bd567a9\"}],\"packageUris\":[\"http://schema.mathworks.com/mf0/Connector/R2020b\"],\"version\":\"1.0\"}"
      mask Display: image('images/z_state.png');
  Subsystem2 : Subsystem
      settings: PortSchema="{\"entries\":[{\"content\":{\"sides\":[{\"content\":{\"connectorIds\":[\"In1\",\"In2\",\"In3\"]},\"type\":\"ConnectorPlacement.EquallySpacedRectSide\",\"uuid\":\"1b79fb4b-1921-4665-8eba-b393f9ea98d6\"},{\"content\":{\"connectorIds\":[\"Out1\"],\"side\":\"RIGHT\"},\"type\":\"ConnectorPlacement.EquallySpacedRectSide\",\"uuid\":\"084d95ac-1716-4b0b-a696-3271535a91cf\"},{\"content\":{\"side\":\"TOP\"},\"type\":\"ConnectorPlacement.EquallySpacedRectSide\",\"uuid\":\"ec91298b-c3b0-4df1-a0b8-53c7de39a879\"},{\"content\":{\"connectorIds\":[\"In4\"],\"side\":\"BOTTOM\"},\"type\":\"ConnectorPlacement.EquallySpacedRectSide\",\"uuid\":\"de14d308-9d82-4371-86bd-ca5ab581d7ed\"}]},\"type\":\"ConnectorPlacement.EquallySpacedConnector\",\"uuid\":\"ce361a1b-48ea-4ff5-b8e2-9f4b10df6d4d\"}],\"packageUris\":[\"http://schema.mathworks.com/mf0/Connector/R2020b\"],\"version\":\"1.0\"}"
      mask Display: image('images/fric_force.png');
  M_clutch : Outport
  wires:
  delta_w/1 -> Gain3/1
  Subsystem1/2(z) -> Subsystem2/3(z)  "z"
  Subsystem1/1(z_dot) -> Subsystem2/2(z_dot)  "z_dot"
  Subsystem2/1(F) -> Gain10/1
  Gain10/1 -> M_clutch/1
  Gain3/1 -> Subsystem/2(v), Subsystem1/1(v), Subsystem2/1(v)  "v"
  " clutch"/1 -> Subsystem2/4(" "), Subsystem1/3(In1), Subsystem/1(N)
  Subsystem/1(g(v)) -> Subsystem1/2(g(v))  "g(v)"

== system printable_simulation/DRIVETRAIN/Transmission/Gearbox/DCT/Dual_Clutch/Clutch1 ==
  " " : Inport
  delta_w : Inport  Port=2
  Bus Selector : BusSelector  OutputSignals=v,z_dot,z
  Bus Selector1 : BusSelector  OutputSignals=-c_cap,c_cap,F
  Gain10 : Gain  Gain=r_eq_clutch
  Gain3 : Gain  Gain=r_eq_clutch
  Scope1 : Scope  NumInputPorts=3
  Scope2 : Scope  NumInputPorts=2
  Scope3 : Scope
  Scope4 : Scope  NumInputPorts=3
  Subsystem : Subsystem
      settings: PortSchema="{\"entries\":[{\"content\":{\"sides\":[{\"content\":{\"connectorIds\":[\"In1\"]},\"type\":\"ConnectorPlacement.EquallySpacedRectSide\",\"uuid\":\"0ae2ed28-5be6-4ce0-b87c-2c13a72d1ad0\"},{\"content\":{\"connectorIds\":[\"In2\",\"Out1\"],\"side\":\"RIGHT\"},\"type\":\"ConnectorPlacement.EquallySpacedRectSide\",\"uuid\":\"8d48d664-ebaf-4c3e-be9e-f793543e8061\"},{\"content\":{\"side\":\"TOP\"},\"type\":\"ConnectorPlacement.EquallySpacedRectSide\",\"uuid\":\"2d66836a-de46-4974-a48b-ee2778be1c08\"},{\"content\":{\"connectorIds\":[\"Out2\"],\"side\":\"BOTTOM\"},\"type\":\"ConnectorPlacement.EquallySpacedRectSide\",\"uuid\":\"e232d9f4-6257-4976-8384-26c462ae0041\"}]},\"type\":\"ConnectorPlacement.EquallySpacedConnector\",\"uuid\":\"ae24f926-3a59-4a74-9cf0-af55dcfbad19\"}],\"packageUris\":[\"http://schema.mathworks.com/mf0/Connector/R2020b\"],\"version\":\"1.0\"}"
      mask Display: image('images/Stribeck.png');
  Subsystem1 : Subsystem
      settings: PortSchema="{\"entries\":[{\"content\":{\"sides\":[{\"content\":{\"connectorIds\":[\"In1\",\"In2\"]},\"type\":\"ConnectorPlacement.EquallySpacedRectSide\",\"uuid\":\"fba00446-fe01-4fd0-a740-7d5efbf0abc7\"},{\"content\":{\"connectorIds\":[\"Out1\",\"Out2\"],\"side\":\"RIGHT\"},\"type\":\"ConnectorPlacement.EquallySpacedRectSide\",\"uuid\":\"28d31996-59d3-4656-988b-c785e0d07c46\"},{\"content\":{\"side\":\"TOP\"},\"type\":\"ConnectorPlacement.EquallySpacedRectSide\",\"uuid\":\"07dfb693-bdac-419f-bf8c-22f11bb5a1ff\"},{\"content\":{\"connectorIds\":[\"In3\"],\"side\":\"BOTTOM\"},\"type\":\"ConnectorPlacement.EquallySpacedRectSide\",\"uuid\":\"e46b7f0d-22dc-4b01-9fc3-2183fe5bd14e\"}]},\"type\":\"ConnectorPlacement.EquallySpacedConnector\",\"uuid\":\"53afe5e8-6f41-4676-b5a4-a094561728b0\"}],\"packageUris\":[\"http://schema.mathworks.com/mf0/Connector/R2020b\"],\"version\":\"1.0\"}"
      mask Display: image('images/z_state.png');
  Subsystem2 : Subsystem
      settings: PortSchema="{\"entries\":[{\"content\":{\"sides\":[{\"content\":{\"connectorIds\":[\"In1\",\"In2\",\"In3\"]},\"type\":\"ConnectorPlacement.EquallySpacedRectSide\",\"uuid\":\"718e9a4c-012a-432e-af1d-56a8c510a1ff\"},{\"content\":{\"connectorIds\":[\"Out1\"],\"side\":\"RIGHT\"},\"type\":\"ConnectorPlacement.EquallySpacedRectSide\",\"uuid\":\"b8acef94-ef29-40e0-b6df-913e21cb4db2\"},{\"content\":{\"connectorIds\":[\"Out2\",\"Out3\"],\"side\":\"TOP\"},\"type\":\"ConnectorPlacement.EquallySpacedRectSide\",\"uuid\":\"42ba6916-bf07-457b-89e7-b10a87e70d96\"},{\"content\":{\"connectorIds\":[\"In4\"],\"side\":\"BOTTOM\"},\"type\":\"ConnectorPlacement.EquallySpacedRectSide\",\"uuid\":\"25c3a005-357f-4967-9fb3-686ba180841f\"}]},\"type\":\"ConnectorPlacement.EquallySpacedConnector\",\"uuid\":\"db3b50fc-f4cd-400b-b8f7-b0301a8ba65b\"}],\"packageUris\":[\"http://schema.mathworks.com/mf0/Connector/R2020b\"],\"version\":\"1.0\"}"
      mask Display: image('images/fric_force.png');
  M_clutch : Outport
  wires:
  Subsystem2/2(Out1) -> Bus Selector/1
  delta_w/1 -> Gain3/1
  Subsystem1/2(z) -> Scope2/1, Subsystem2/3(z)  "z"
  Subsystem1/1(z_dot) -> Scope2/2, Subsystem2/2(z_dot)  "z_dot"
  Subsystem2/1(F) -> Gain10/1  "c2_F"
  Gain10/1 -> M_clutch/1  "M_clutch"
  Gain3/1 -> Subsystem2/1(v), Scope3/1, Subsystem1/1(v), Subsystem/2(v)  "v"
  Subsystem/1(g(v)) -> Subsystem1/2(g(v))  "g(v)"
  " "/1 -> Subsystem2/4(clutch), Subsystem1/3("clutch "), Subsystem/1(N)
  Bus Selector/2 -> Scope4/2  "<z_dot>"
  Bus Selector/3 -> Scope4/3  "<z>"
  Bus Selector/1 -> Scope4/1  "<v>"
  Subsystem2/3(Out2) -> Bus Selector1/1
  Bus Selector1/1 -> Scope1/1  "<-c_cap>"
  Bus Selector1/2 -> Scope1/2  "<c_cap>"
  Bus Selector1/3 -> Scope1/3  "<F>"

== system printable_simulation/DRIVETRAIN/Transmission/Gearbox/DCT/Dual_Clutch/Clutch2 ==
  " " : Inport
  delta_w : Inport  Port=2
  Bus Selector : BusSelector  OutputSignals=v,z_dot,z
  Bus Selector1 : BusSelector  OutputSignals=-c_cap,c_cap,F
  Gain10 : Gain  Gain=r_eq_clutch
  Gain3 : Gain  Gain=r_eq_clutch
  Scope1 : Scope  NumInputPorts=3
  Scope2 : Scope  NumInputPorts=2
  Scope3 : Scope
  Scope4 : Scope  NumInputPorts=3
  Subsystem : Subsystem
      settings: PortSchema="{\"entries\":[{\"content\":{\"sides\":[{\"content\":{\"connectorIds\":[\"In1\"]},\"type\":\"ConnectorPlacement.EquallySpacedRectSide\",\"uuid\":\"0ae2ed28-5be6-4ce0-b87c-2c13a72d1ad0\"},{\"content\":{\"connectorIds\":[\"In2\",\"Out1\"],\"side\":\"RIGHT\"},\"type\":\"ConnectorPlacement.EquallySpacedRectSide\",\"uuid\":\"8d48d664-ebaf-4c3e-be9e-f793543e8061\"},{\"content\":{\"side\":\"TOP\"},\"type\":\"ConnectorPlacement.EquallySpacedRectSide\",\"uuid\":\"2d66836a-de46-4974-a48b-ee2778be1c08\"},{\"content\":{\"connectorIds\":[\"Out2\"],\"side\":\"BOTTOM\"},\"type\":\"ConnectorPlacement.EquallySpacedRectSide\",\"uuid\":\"e232d9f4-6257-4976-8384-26c462ae0041\"}]},\"type\":\"ConnectorPlacement.EquallySpacedConnector\",\"uuid\":\"ae24f926-3a59-4a74-9cf0-af55dcfbad19\"}],\"packageUris\":[\"http://schema.mathworks.com/mf0/Connector/R2020b\"],\"version\":\"1.0\"}"
      mask Display: image('images/Stribeck.png');
  Subsystem1 : Subsystem
      settings: PortSchema="{\"entries\":[{\"content\":{\"sides\":[{\"content\":{\"connectorIds\":[\"In1\",\"In2\"]},\"type\":\"ConnectorPlacement.EquallySpacedRectSide\",\"uuid\":\"fba00446-fe01-4fd0-a740-7d5efbf0abc7\"},{\"content\":{\"connectorIds\":[\"Out1\",\"Out2\"],\"side\":\"RIGHT\"},\"type\":\"ConnectorPlacement.EquallySpacedRectSide\",\"uuid\":\"28d31996-59d3-4656-988b-c785e0d07c46\"},{\"content\":{\"side\":\"TOP\"},\"type\":\"ConnectorPlacement.EquallySpacedRectSide\",\"uuid\":\"07dfb693-bdac-419f-bf8c-22f11bb5a1ff\"},{\"content\":{\"connectorIds\":[\"In3\"],\"side\":\"BOTTOM\"},\"type\":\"ConnectorPlacement.EquallySpacedRectSide\",\"uuid\":\"e46b7f0d-22dc-4b01-9fc3-2183fe5bd14e\"}]},\"type\":\"ConnectorPlacement.EquallySpacedConnector\",\"uuid\":\"53afe5e8-6f41-4676-b5a4-a094561728b0\"}],\"packageUris\":[\"http://schema.mathworks.com/mf0/Connector/R2020b\"],\"version\":\"1.0\"}"
      mask Display: image('images/z_state.png');
  Subsystem2 : Subsystem
      settings: PortSchema="{\"entries\":[{\"content\":{\"sides\":[{\"content\":{\"connectorIds\":[\"In1\",\"In2\",\"In3\"]},\"type\":\"ConnectorPlacement.EquallySpacedRectSide\",\"uuid\":\"718e9a4c-012a-432e-af1d-56a8c510a1ff\"},{\"content\":{\"connectorIds\":[\"Out1\"],\"side\":\"RIGHT\"},\"type\":\"ConnectorPlacement.EquallySpacedRectSide\",\"uuid\":\"b8acef94-ef29-40e0-b6df-913e21cb4db2\"},{\"content\":{\"connectorIds\":[\"Out2\",\"Out3\"],\"side\":\"TOP\"},\"type\":\"ConnectorPlacement.EquallySpacedRectSide\",\"uuid\":\"42ba6916-bf07-457b-89e7-b10a87e70d96\"},{\"content\":{\"connectorIds\":[\"In4\"],\"side\":\"BOTTOM\"},\"type\":\"ConnectorPlacement.EquallySpacedRectSide\",\"uuid\":\"25c3a005-357f-4967-9fb3-686ba180841f\"}]},\"type\":\"ConnectorPlacement.EquallySpacedConnector\",\"uuid\":\"db3b50fc-f4cd-400b-b8f7-b0301a8ba65b\"}],\"packageUris\":[\"http://schema.mathworks.com/mf0/Connector/R2020b\"],\"version\":\"1.0\"}"
      mask Display: image('images/fric_force.png');
  M_clutch : Outport
  wires:
  Subsystem2/2(Out1) -> Bus Selector/1
  delta_w/1 -> Gain3/1
  Subsystem1/2(z) -> Scope2/1, Subsystem2/3(z)  "z"
  Subsystem1/1(z_dot) -> Scope2/2, Subsystem2/2(z_dot)  "z_dot"
  Subsystem2/1(F) -> Gain10/1  "c2_F"
  Gain10/1 -> M_clutch/1  "M_clutch"
  Gain3/1 -> Subsystem2/1(v), Scope3/1, Subsystem1/1(v), Subsystem/2(v)  "v"
  Subsystem/1(g(v)) -> Subsystem1/2(g(v))  "g(v)"
  " "/1 -> Subsystem2/4(clutch), Subsystem1/3("clutch "), Subsystem/1(N)
  Bus Selector/2 -> Scope4/2  "<z_dot>"
  Bus Selector/3 -> Scope4/3  "<z>"
  Bus Selector/1 -> Scope4/1  "<v>"
  Subsystem2/3(Out2) -> Bus Selector1/1
  Bus Selector1/1 -> Scope1/1  "<-c_cap>"
  Bus Selector1/2 -> Scope1/2  "<c_cap>"
  Bus Selector1/3 -> Scope1/3  "<F>"

== system printable_simulation/DRIVETRAIN/Transmission/Gearbox/DCT/Stage_2.1/Nothing ==
  Torque_in : Inport
  Speed_fdbk : Inport  Port=2
  Torque_out : Outport
  Speed_out : Outport  Port=2
  wires:
  Torque_in/1 -> Torque_out/1  "T_Rotor"
  Speed_fdbk/1 -> Speed_out/1

== system printable_simulation/DRIVETRAIN/Transmission/Gearbox/DCT/Stage_2.1/Spur ==
  Torque_in : Inport
  Speed_fdbk : Inport  Port=2
  Spur2 : Subsystem  mask{i=Stage2.i1, J1=Stage2.Spur11.J, J2=Stage2.Spur12.J}
      mask prompts: i "Ratio"; J1 "Input_Gear_Inertia"; J2 "Output_Gear_Inertia"
      settings: PortSchema="{\"entries\":[{\"content\":{\"sides\":[{\"content\":{\"connectorIds\":[\"In1\",\"Out2\"]},\"type\":\"ConnectorPlacement.EquallySpacedRectSide\",\"uuid\":\"898fedf9-82f7-4bc2-bf05-880de36b191d\"},{\"content\":{\"connectorIds\":[\"Out1\",\"In2\"],\"side\":\"RIGHT\"},\"type\":\"ConnectorPlacement.EquallySpacedRectSide\",\"uuid\":\"50317b6c-245f-4bd1-a8cd-7a774957ae86\"},{\"content\":{\"side\":\"TOP\"},\"type\":\"ConnectorPlacement.EquallySpacedRectSide\",\"uuid\":\"ff1de2a1-7305-40d8-9e1f-fd0fa1e7d830\"}]},\"type\":\"ConnectorPlacement.EquallySpacedConnector\",\"uuid\":\"6ce82d73-f3da-4f59-9039-464a6ef3e9c5\"}],\"packageUris\":[\"http://schema.mathworks.com/mf0/Connector/R2020b\"],\"version\":\"1.0\"}"
  Torque_out : Outport
  Speed_out : Outport  Port=2
  wires:
  Speed_fdbk/1 -> Spur2/2(Speed_fdbk)
  Torque_in/1 -> Spur2/1(Torque_in)
  Spur2/2(phi_dot) -> Speed_out/1
  Spur2/1(Torque_out) -> Torque_out/1

== system printable_simulation/DRIVETRAIN/Transmission/Gearbox/DCT/Stage_2.2/Nothing ==
  Torque_in : Inport
  Speed_fdbk : Inport  Port=2
  Torque_out : Outport
  Speed_out : Outport  Port=2
  wires:
  Torque_in/1 -> Torque_out/1  "T_Rotor"
  Speed_fdbk/1 -> Speed_out/1

== system printable_simulation/DRIVETRAIN/Transmission/Gearbox/DCT/Stage_2.2/Spur ==
  Torque_in : Inport
  Speed_fdbk : Inport  Port=2
  Spur2 : Subsystem  mask{i=Stage2.i2, J1=Stage2.Spur21.J, J2=Stage2.Spur22.J}
      mask prompts: i "Ratio"; J1 "Input_Gear_Inertia"; J2 "Output_Gear_Inertia"
      settings: PortSchema="{\"entries\":[{\"content\":{\"sides\":[{\"content\":{\"connectorIds\":[\"In1\",\"Out2\"]},\"type\":\"ConnectorPlacement.EquallySpacedRectSide\",\"uuid\":\"898fedf9-82f7-4bc2-bf05-880de36b191d\"},{\"content\":{\"connectorIds\":[\"Out1\",\"In2\"],\"side\":\"RIGHT\"},\"type\":\"ConnectorPlacement.EquallySpacedRectSide\",\"uuid\":\"50317b6c-245f-4bd1-a8cd-7a774957ae86\"},{\"content\":{\"side\":\"TOP\"},\"type\":\"ConnectorPlacement.EquallySpacedRectSide\",\"uuid\":\"ff1de2a1-7305-40d8-9e1f-fd0fa1e7d830\"}]},\"type\":\"ConnectorPlacement.EquallySpacedConnector\",\"uuid\":\"6ce82d73-f3da-4f59-9039-464a6ef3e9c5\"}],\"packageUris\":[\"http://schema.mathworks.com/mf0/Connector/R2020b\"],\"version\":\"1.0\"}"
  Torque_out : Outport
  Speed_out : Outport  Port=2
  wires:
  Torque_in/1 -> Spur2/1(Torque_in)
  Spur2/2(phi_dot) -> Speed_out/1
  Spur2/1(Torque_out) -> Torque_out/1
  Speed_fdbk/1 -> Spur2/2(Speed_fdbk)

== system printable_simulation/DRIVETRAIN/Transmission/Gearbox/DCT/Stage_3/Nothing ==
  Torque_in : Inport
  Speed_fdbk : Inport  Port=2
  Torque_out : Outport
  Speed_out : Outport  Port=2
  wires:
  Speed_fdbk/1 -> Speed_out/1
  Torque_in/1 -> Torque_out/1

== system printable_simulation/DRIVETRAIN/Transmission/Gearbox/DCT/Stage_3/Spur ==
  Torque_in : Inport
  Speed_fdbk : Inport  Port=2
  Shaft : Subsystem  mask{J=Shaft.J}
      mask prompts: J "Inertia_kgm^2"
      settings: PortSchema="{\"entries\":[{\"content\":{\"sides\":[{\"content\":{\"connectorIds\":[\"In1\",\"Out2\"]},\"type\":\"ConnectorPlacement.EquallySpacedRectSide\",\"uuid\":\"898fedf9-82f7-4bc2-bf05-880de36b191d\"},{\"content\":{\"connectorIds\":[\"Out1\",\"In2\"],\"side\":\"RIGHT\"},\"type\":\"ConnectorPlacement.EquallySpacedRectSide\",\"uuid\":\"50317b6c-245f-4bd1-a8cd-7a774957ae86\"},{\"content\":{\"side\":\"TOP\"},\"type\":\"ConnectorPlacement.EquallySpacedRectSide\",\"uuid\":\"ff1de2a1-7305-40d8-9e1f-fd0fa1e7d830\"}]},\"type\":\"ConnectorPlacement.EquallySpacedConnector\",\"uuid\":\"6ce82d73-f3da-4f59-9039-464a6ef3e9c5\"}],\"packageUris\":[\"http://schema.mathworks.com/mf0/Connector/R2020b\"],\"version\":\"1.0\"}"
  Spur3 : Subsystem  mask{i=Stage3.i, J1=Stage3.Spur1.J, J2=Stage3.Spur2.J}
      mask prompts: i "Ratio"; J1 "Input_Gear_Inertia"; J2 "Output_Gear_Inertia"
      settings: PortSchema="{\"entries\":[{\"content\":{\"sides\":[{\"content\":{\"connectorIds\":[\"In1\",\"Out2\"]},\"type\":\"ConnectorPlacement.EquallySpacedRectSide\",\"uuid\":\"898fedf9-82f7-4bc2-bf05-880de36b191d\"},{\"content\":{\"connectorIds\":[\"Out1\",\"In2\"],\"side\":\"RIGHT\"},\"type\":\"ConnectorPlacement.EquallySpacedRectSide\",\"uuid\":\"50317b6c-245f-4bd1-a8cd-7a774957ae86\"},{\"content\":{\"side\":\"TOP\"},\"type\":\"ConnectorPlacement.EquallySpacedRectSide\",\"uuid\":\"ff1de2a1-7305-40d8-9e1f-fd0fa1e7d830\"}]},\"type\":\"ConnectorPlacement.EquallySpacedConnector\",\"uuid\":\"6ce82d73-f3da-4f59-9039-464a6ef3e9c5\"}],\"packageUris\":[\"http://schema.mathworks.com/mf0/Connector/R2020b\"],\"version\":\"1.0\"}"
  Torque_out : Outport
  Speed_out : Outport  Port=2
  wires:
  Speed_fdbk/1 -> Spur3/2(Speed_fdbk)
  Spur3/2(phi_dot) -> Shaft/2(Speed_fdbk)
  Spur3/1(Torque_out) -> Torque_out/1
  Torque_in/1 -> Shaft/1(Torque_in)
  Shaft/2(phi_dot) -> Speed_out/1
  Shaft/1(Torque_out) -> Spur3/1(Torque_in)

== system printable_simulation/DRIVETRAIN/Transmission/Gearbox/AMT/Clutch/LuGre Model/Subsystem ==
  N : Inport
  v : Inport  Port=2
  Abs : Abs  SaturateOnIntegerOverflow=off
  Constant1 : Constant  Value=vs
  Divide1 : Product  Inputs=/*
  Divide2 : Product  Inputs=/*
  Exp : Math
  Gain1 : Gain  Gain=n_surfaces
  Gain4 : Gain  Gain=mi_s
  Gain5 : Gain  Gain=1/sigma0
  Gain6 : Gain  Gain=mi_c
  Gain7 : Gain  Gain=N_clutch*2
  Square : Math  Operator=square
  Sum4 : Sum  Inputs=+|+
  Sum5 : Sum  Inputs=|+-
  g(v) : Outport
  wires:
  Gain1/1 -> Gain4/1, Gain6/1
  Gain4/1 -> Sum5/1  "Fs"
  Abs/1 -> Gain7/1
  v/1 -> Divide1/2
  N/1 -> Abs/1
  Gain5/1 -> g(v)/1  "g(v)"
  Square/1 -> Exp/1
  Divide1/1 -> Square/1
  Constant1/1 -> Divide1/1
  Gain7/1 -> Gain1/1  "Fn"
  Exp/1 -> Divide2/1
  Gain6/1 -> Sum5/2, Sum4/2  "Fc"
  Divide2/1 -> Sum4/1
  Sum5/1 -> Divide2/2
  Sum4/1 -> Gain5/1

== system printable_simulation/DRIVETRAIN/Transmission/Gearbox/AMT/Clutch/LuGre Model/Subsystem1 ==
  v : Inport
  g(v) : Inport  Port=2
  In1 : Inport  Port=3
  Abs1 : Abs  SaturateOnIntegerOverflow=off
  Divide : Product  Inputs=*/
  Integrator : Integrator
  Product2 : Product
  Saturation : Saturate  UpperLimit=inf  LowerLimit=0.01
  Sum2 : Sum  Inputs=|+-
  Switch : Switch  Criteria=u2 ~= 0  SaturateOnIntegerOverflow=off  InputSameDT=off
  z_dot : Outport
  z : Outport  Port=2
  wires:
  In1/1 -> Switch/2, Switch/3
  g(v)/1 -> Saturation/1
  Product2/1 -> Sum2/2
  Abs1/1 -> Divide/1
  Saturation/1 -> Divide/2
  Sum2/1 -> z_dot/1, Integrator/1  "z_dot"
  Switch/1 -> Abs1/1, Sum2/1
  Divide/1 -> Product2/1
  Integrator/1 -> Product2/2, z/1  "z"
  v/1 -> Switch/1

== system printable_simulation/DRIVETRAIN/Transmission/Gearbox/AMT/Clutch/LuGre Model/Subsystem2 ==
  v : Inport
  z_dot : Inport  Port=2
  z : Inport  Port=3
  " " : Inport  Port=4
  Gain : Gain  Gain=sigma2
  Gain1 : Gain  Gain=sigma1
  Gain2 : Gain  Gain=sigma0
  Scope : Scope  NumInputPorts=3
  Sum3 : Sum  Inputs=+++
  Switch : Switch  Criteria=u2 ~= 0  SaturateOnIntegerOverflow=off  InputSameDT=off
  F : Outport
  wires:
  z/1 -> Gain2/1
  z_dot/1 -> Gain1/1
  Gain1/1 -> Sum3/2, Scope/2
  Sum3/1 -> Switch/1  "F"
  Gain2/1 -> Sum3/3, Scope/1
  Gain/1 -> Sum3/1, Scope/3
  v/1 -> Gain/1
  " "/1 -> Switch/2, Switch/3
  Switch/1 -> F/1

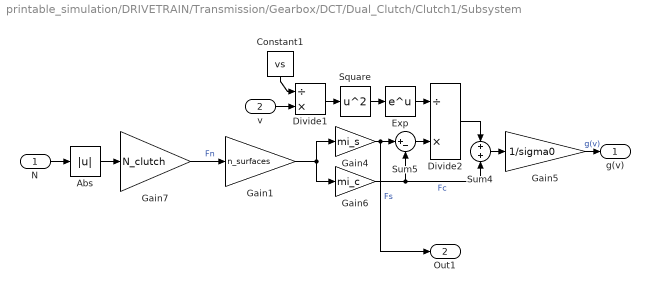
== system printable_simulation/DRIVETRAIN/Transmission/Gearbox/DCT/Dual_Clutch/Clutch1/Subsystem ==
  N : Inport
  v : Inport  Port=2
  Abs : Abs  SaturateOnIntegerOverflow=off
  Constant1 : Constant  Value=vs
  Divide1 : Product  Inputs=/*
  Divide2 : Product  Inputs=/*
  Exp : Math
  Gain1 : Gain  Gain=n_surfaces
  Gain4 : Gain  Gain=mi_s
  Gain5 : Gain  Gain=1/sigma0
  Gain6 : Gain  Gain=mi_c
  Gain7 : Gain  Gain=N_clutch
  Square : Math  Operator=square
  Sum4 : Sum  Inputs=+|+
  Sum5 : Sum  Inputs=|+-
  g(v) : Outport
  Out1 : Outport  Port=2
  wires:
  Gain1/1 -> Gain6/1, Gain4/1
  Gain4/1 -> Out1/1, Sum5/1  "Fs"
  Abs/1 -> Gain7/1
  v/1 -> Divide1/2
  N/1 -> Abs/1
  Gain5/1 -> g(v)/1  "g(v)"
  Square/1 -> Exp/1
  Divide1/1 -> Square/1
  Constant1/1 -> Divide1/1
  Gain7/1 -> Gain1/1  "Fn"
  Exp/1 -> Divide2/1
  Gain6/1 -> Sum5/2, Sum4/2  "Fc"
  Divide2/1 -> Sum4/1
  Sum5/1 -> Divide2/2
  Sum4/1 -> Gain5/1

== system printable_simulation/DRIVETRAIN/Transmission/Gearbox/DCT/Dual_Clutch/Clutch1/Subsystem1 ==
  v : Inport
  g(v) : Inport  Port=2
  "clutch " : Inport  Port=3
  Abs1 : Abs  SaturateOnIntegerOverflow=off
  Compare To Constant : simulink/Logic and Bit Operations/Compare To Constant  relop=<=  const=0.001  OutDataTypeStr=boolean
  Divide : Product  Inputs=*/
  Integrator : Integrator  ExternalReset=level
  Product2 : Product
  Saturation : Saturate  UpperLimit=inf  LowerLimit=0.000001
  Scope : Scope  NumInputPorts=2
  Sum2 : Sum  Inputs=|+-
  z_dot : Outport
  z : Outport  Port=2
  wires:
  Compare To Constant/1 -> Integrator/2
  g(v)/1 -> Saturation/1, Scope/2
  Product2/1 -> Sum2/2
  Abs1/1 -> Divide/1
  Saturation/1 -> Divide/2, Scope/1
  Sum2/1 -> z_dot/1, Integrator/1  "z_dot"
  v/1 -> Sum2/1, Abs1/1
  Divide/1 -> Product2/1
  Integrator/1 -> z/1, Product2/2  "z"
  "clutch "/1 -> Compare To Constant/1
